simulink model "fm_demod_fixed"  (R2021b)
settings: Solver=FixedStepDiscrete  StartTime=0  StopTime=30  FixedStep=4e-06  RelTol=1e-3
libraries: dspmlti4 x1
settings Model: FPTRunName=FloatingPoint_Baseline  Creator=caccolillo  LastModifiedBy=caccolillo
settings DataIOCC: ReturnWorkspaceOutputs=off
settings DebuggingCC: SingleTaskRateTransMsg=error
settings HardwareCC: ProdBitPerPointer=32  ProdBitPerSizeT=32  ProdBitPerPtrDiffT=32  ProdLargestAtomicFloat=None  ProdIntDivRoundTo=Undefined  ProdEndianess=Unspecified  ProdWordSize=32  ProdHWDeviceType=ASIC/FPGA->ASIC/FPGA  TargetBitPerLong=64  TargetBitPerPointer=64  TargetBitPerSizeT=64  TargetBitPerPtrDiffT=64  TargetLongLongMode=on  TargetIntDivRoundTo=Zero  TargetEndianess=LittleEndian  TargetWordSize=64  TargetHWDeviceType=Custom Processor->MATLAB Host Computer  ProdEqTarget=off

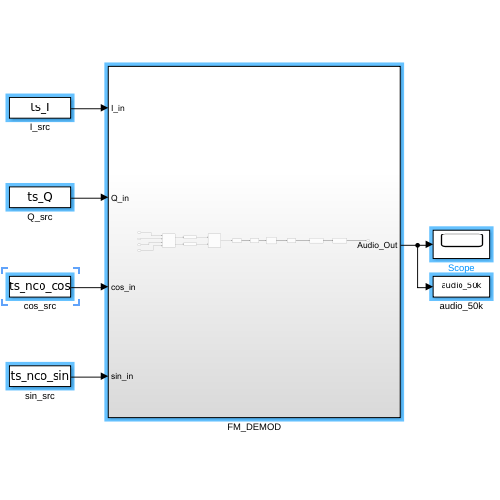
[thumbnail: Simulink's stored preview of the top-level diagram]
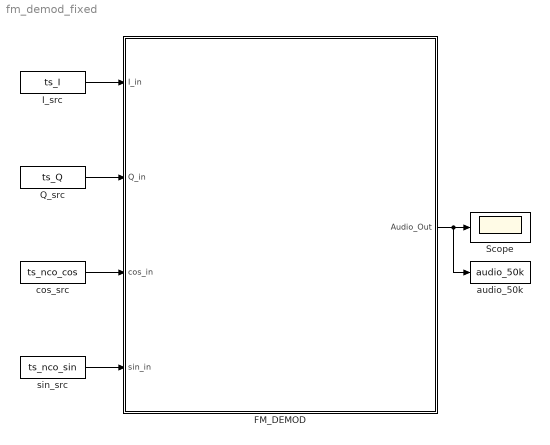
== system fm_demod_fixed ==
  FM_DEMOD : Subsystem
  I_src : FromWorkspace  VariableName=ts_I  OutDataTypeStr=fixdt(1,16,15)  SampleTime=4e-06  Interpolate=off  OutputAfterFinalValue=Holding final value
  Q_src : FromWorkspace  VariableName=ts_Q  OutDataTypeStr=fixdt(1,16,15)  SampleTime=4e-06  Interpolate=off  OutputAfterFinalValue=Holding final value
  Scope : Scope
  audio_50k : ToWorkspace  VariableName=audio_50k  SampleTime=2e-05
  cos_src : FromWorkspace  VariableName=ts_nco_cos  OutDataTypeStr=fixdt(1,16,15)  SampleTime=4e-06  Interpolate=off  OutputAfterFinalValue=Holding final value
  sin_src : FromWorkspace  VariableName=ts_nco_sin  OutDataTypeStr=fixdt(1,16,15)  SampleTime=4e-06  Interpolate=off  OutputAfterFinalValue=Holding final value
  wires:
  FM_DEMOD/1(Audio_Out) -> audio_50k/1, Scope/1
  I_src/1 -> FM_DEMOD/1(I_in)
  Q_src/1 -> FM_DEMOD/2(Q_in)
  sin_src/1 -> FM_DEMOD/4(sin_in)
  cos_src/1 -> FM_DEMOD/3(cos_in)

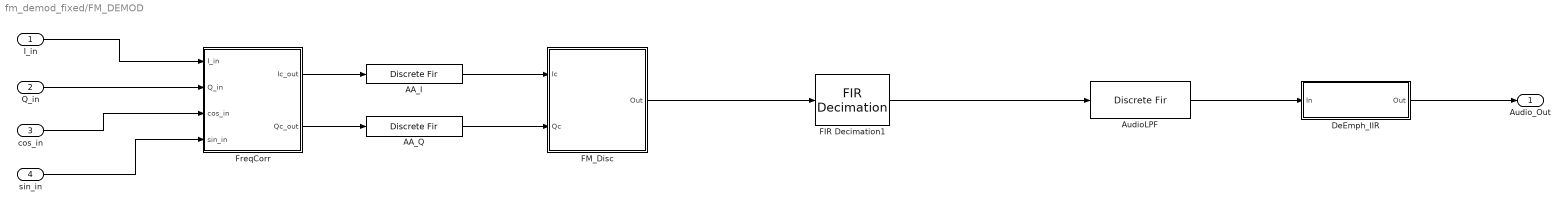
== system fm_demod_fixed/FM_DEMOD ==
  I_in : Inport
  Q_in : Inport  Port=2
  cos_in : Inport  Port=3
  sin_in : Inport  Port=4
  AA_I : DiscreteFir  Coefficients=[-6.83735984948204e-06 1.75449332456455e-05 -2.57498904954935e-05 2.22172761459078e-05 -2.99370071174519e-19 -3.92649348170435e-05 8.15857314818403e-05 -0.000102971543129532 7.91656098368774e-05 -3.24330107466436e-18 -0.000118229493833425 0.000230339323629204 -0.000275024861244747 0.000201424428805084 -1.97573802370049e-18 -0.000277296850682596 0.000521831881485624 -0.000603748721149827 0.000429629869716551 -3.69375267985403e-18 -0.00056213481227273 0.00103420375089876 -0.00117166952626484 0.000817594936231136 -6.1350079045508e-18 -0.00103254111923509 0.00186942750628691 -0.0020862979168 0.00143542734292027 -9.30071338109499e-18 -0.00176688426495698 0.00316197088837946 -0.00349061204586083 0.00237738739067954 -1.30795303176458e-17 -0.00287369810390145 0.00510160254853362 -0.00559079244160399 0.0037827464698203 -1.724148644289e-17 -0.00452266933996601 0.00799466321850092 -0.00873128617137548 0.0058928045310547 -2.14546833372083e-17 -0.00703185352755392 0.0124399916379781 -0.0136155611823128 0.00922338626974311 -2.53243457513243e-17 -0.0111510442447546 0.0199262698383597 -0.0220945427009549 0.0152176990921621 -2.84485240246462e-17 -0.0192996698147462 0.0356852825814448 -0.0413494048380904 0.0301723992042311 -3.04804610369061e-17 -0.0460953947614038 0.100083939525413 -0.150813546567284 0.186927410503456 0.800001561488201 0.186927410503456 -0.150813546567284 0.100083939525413 -0.0460953947614038 -3.04804610369061e-17 0.0301723992042311 -0.0413494048380904 0.0356852825814448 -0.0192996698147462 -2.84485240246462e-17 0.0152176990921621 -0.0220945427009549 0.0199262698383597 -0.0111510442447546 -2.53243457513243e-17 0.00922338626974311 -0.0136155611823128 0.0124399916379781 -0.00703185352755392 -2.14546833372083e-17 0.0058928045310547 -0.00873128617137548 0.00799466321850092 -0.00452266933996601 -1.724148644289e-17 0.0037827464698203 -0.00559079244160399 0.00510160254853362 -0.00287369810390145 -1.30795303176458e-17 0.00237738739067954 -0.00349061204586083 0.00316197088837946 -0.00176688426495698 -9.30071338109499e-18 0.00143542734292027 -0.0020862979168 0.00186942750628691 -0.00103254111923509 -6.1350079045508e-18 0.000817594936231136 -0.00117166952626484 0.00103420375089876 -0.00056213481227273 -3.69375267985403e-18 0.000429629869716551 -0.000603748721149827 0.000521831881485624 -0.000277296850682596 -1.97573802370049e-18 0.000201424428805084 -0.000275024861244747 0.000230339323629204 -0.000118229493833425 -3.24330107466436e-18 7.91656098368774e-05 -0.000102971543129532 8.15857314818403e-05 -3.92649348170435e-05 -2.99370071174519e-19 2.22172761459078e-05 -2.57498904954935e-05 1.75449332456455e-05 -6.83735984948204e-06]  SampleTime=4e-06  CoefDataTypeStr=fixdt(1,32,30)  OutDataTypeStr=fixdt(1,18,17)  SaturateOnIntegerOverflow=on
  AA_Q : DiscreteFir  Coefficients=[-6.83735984948204e-06 1.75449332456455e-05 -2.57498904954935e-05 2.22172761459078e-05 -2.99370071174519e-19 -3.92649348170435e-05 8.15857314818403e-05 -0.000102971543129532 7.91656098368774e-05 -3.24330107466436e-18 -0.000118229493833425 0.000230339323629204 -0.000275024861244747 0.000201424428805084 -1.97573802370049e-18 -0.000277296850682596 0.000521831881485624 -0.000603748721149827 0.000429629869716551 -3.69375267985403e-18 -0.00056213481227273 0.00103420375089876 -0.00117166952626484 0.000817594936231136 -6.1350079045508e-18 -0.00103254111923509 0.00186942750628691 -0.0020862979168 0.00143542734292027 -9.30071338109499e-18 -0.00176688426495698 0.00316197088837946 -0.00349061204586083 0.00237738739067954 -1.30795303176458e-17 -0.00287369810390145 0.00510160254853362 -0.00559079244160399 0.0037827464698203 -1.724148644289e-17 -0.00452266933996601 0.00799466321850092 -0.00873128617137548 0.0058928045310547 -2.14546833372083e-17 -0.00703185352755392 0.0124399916379781 -0.0136155611823128 0.00922338626974311 -2.53243457513243e-17 -0.0111510442447546 0.0199262698383597 -0.0220945427009549 0.0152176990921621 -2.84485240246462e-17 -0.0192996698147462 0.0356852825814448 -0.0413494048380904 0.0301723992042311 -3.04804610369061e-17 -0.0460953947614038 0.100083939525413 -0.150813546567284 0.186927410503456 0.800001561488201 0.186927410503456 -0.150813546567284 0.100083939525413 -0.0460953947614038 -3.04804610369061e-17 0.0301723992042311 -0.0413494048380904 0.0356852825814448 -0.0192996698147462 -2.84485240246462e-17 0.0152176990921621 -0.0220945427009549 0.0199262698383597 -0.0111510442447546 -2.53243457513243e-17 0.00922338626974311 -0.0136155611823128 0.0124399916379781 -0.00703185352755392 -2.14546833372083e-17 0.0058928045310547 -0.00873128617137548 0.00799466321850092 -0.00452266933996601 -1.724148644289e-17 0.0037827464698203 -0.00559079244160399 0.00510160254853362 -0.00287369810390145 -1.30795303176458e-17 0.00237738739067954 -0.00349061204586083 0.00316197088837946 -0.00176688426495698 -9.30071338109499e-18 0.00143542734292027 -0.0020862979168 0.00186942750628691 -0.00103254111923509 -6.1350079045508e-18 0.000817594936231136 -0.00117166952626484 0.00103420375089876 -0.00056213481227273 -3.69375267985403e-18 0.000429629869716551 -0.000603748721149827 0.000521831881485624 -0.000277296850682596 -1.97573802370049e-18 0.000201424428805084 -0.000275024861244747 0.000230339323629204 -0.000118229493833425 -3.24330107466436e-18 7.91656098368774e-05 -0.000102971543129532 8.15857314818403e-05 -3.92649348170435e-05 -2.99370071174519e-19 2.22172761459078e-05 -2.57498904954935e-05 1.75449332456455e-05 -6.83735984948204e-06]  SampleTime=4e-06  CoefDataTypeStr=fixdt(1,32,30)  OutDataTypeStr=fixdt(1,18,17)  SaturateOnIntegerOverflow=on
  AudioLPF : DiscreteFir  Coefficients=[1.10630118570443e-05 -1.08432976692692e-05 -1.59142086028176e-05 3.59480844718192e-05 -2.24526157623805e-19 -6.3531604158573e-05 5.04224416038869e-05 6.36395179157821e-05 -0.000128091851178763 8.0856679998092e-20 0.000191298150298555 -0.000142356645994619 -0.000169973655366647 0.00032590954596866 -4.34759523472029e-18 -0.000448672940221937 0.000322507834315517 0.000373134910757946 -0.0006951514104051 5.74683897466055e-18 0.000909547578353881 -0.000639169095981201 -0.00072412708930962 0.00132288817217507 -4.60122732508374e-18 -0.00167067624001808 0.00115536255612823 0.00128939500777255 -0.00232255579115897 -2.66068793726318e-18 0.00285886102290262 -0.00195419333229843 -0.00215730347509865 0.00384666968989025 -9.80958675736531e-18 -0.00464971230078449 0.00315294417194669 0.00345527827337028 -0.00612057431070915 3.79397487923056e-17 0.00731778722123629 -0.00494094288248589 -0.00539619807418157 0.00953469874826618 -1.60909124744493e-17 -0.0113777072824711 0.00768828985811575 0.00841482727616552 -0.0149236597035326 1.89931412434575e-17 0.0180426564366787 -0.0123150354732263 -0.0136550934687819 0.0246226012963577 -2.13362603825508e-17 -0.0312273276085871 0.0220545804321383 0.025555178741863 -0.0488196639492607 2.28602036682186e-17 0.0745834518040139 -0.0618548918364519 -0.0932073183232599 0.302453023437542 0.599997441258177 0.302453023437542 -0.0932073183232599 -0.0618548918364519 0.0745834518040139 2.28602036682186e-17 -0.0488196639492607 0.025555178741863 0.0220545804321383 -0.0312273276085871 -2.13362603825508e-17 0.0246226012963577 -0.0136550934687819 -0.0123150354732263 0.0180426564366787 1.89931412434575e-17 -0.0149236597035326 0.00841482727616552 0.00768828985811575 -0.0113777072824711 -1.60909124744493e-17 0.00953469874826618 -0.00539619807418157 -0.00494094288248589 0.00731778722123629 3.79397487923056e-17 -0.00612057431070915 0.00345527827337028 0.00315294417194669 -0.00464971230078449 -9.80958675736531e-18 0.00384666968989025 -0.00215730347509865 -0.00195419333229843 0.00285886102290262 -2.66068793726318e-18 -0.00232255579115897 0.00128939500777255 0.00115536255612823 -0.00167067624001808 -4.60122732508374e-18 0.00132288817217507 -0.00072412708930962 -0.000639169095981201 0.000909547578353881 5.74683897466055e-18 -0.0006951514104051 0.000373134910757946 0.000322507834315517 -0.000448672940221937 -4.34759523472029e-18 0.00032590954596866 -0.000169973655366647 -0.000142356645994619 0.000191298150298555 8.0856679998092e-20 -0.000128091851178763 6.36395179157821e-05 5.04224416038869e-05 -6.3531604158573e-05 -2.24526157623805e-19 3.59480844718192e-05 -1.59142086028176e-05 -1.08432976692692e-05 1.10630118570443e-05]  SampleTime=2e-05  CoefDataTypeStr=fixdt(1,32,14)  AccumDataTypeStr=fixdt(1,40,14)  OutDataTypeStr=fixdt(1,32,14)  SaturateOnIntegerOverflow=on
  DeEmph_IIR : Subsystem
  FIR Decimation1 : dspmlti4/FIR Decimation  FilterSource=Dialog parameters  h=fir1(40, 1/5)  D=5  filtStruct=Direct form transposed  FilterObject=FDECIM  framing=Enforce single-rate processing  inputOffset=0  outputBufInitCond=0  roundingMode=Floor  overflowMode=off  firstCoeffDataTypeStr=Inherit: Same word length as input  firstCoeffMin=[]  firstCoeffMax=[]  firstCoeffLastDataTypeStr=Inherit: Same word length as input  outputDataTypeStr=Inherit: Same as accumulator  outputMin=[]  outputMax=[]  outputLastDataTypeStr=Inherit: Same as accumulator
  FM_Disc : Subsystem
  FreqCorr : Subsystem
  Audio_Out : Outport
  wires:
  Q_in/1 -> FreqCorr/2(Q_in)
  FreqCorr/2(Qc_out) -> AA_Q/1
  cos_in/1 -> FreqCorr/3(cos_in)
  AA_Q/1 -> FM_Disc/2(Qc)
  sin_in/1 -> FreqCorr/4(sin_in)
  I_in/1 -> FreqCorr/1(I_in)
  FM_Disc/1(Out) -> FIR Decimation1/1
  FreqCorr/1(Ic_out) -> AA_I/1
  AA_I/1 -> FM_Disc/1(Ic)
  FIR Decimation1/1 -> AudioLPF/1
  AudioLPF/1 -> DeEmph_IIR/1(In)
  DeEmph_IIR/1(Out) -> Audio_Out/1

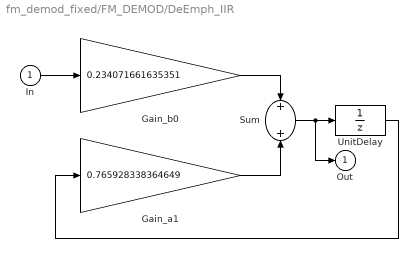
== system fm_demod_fixed/FM_DEMOD/DeEmph_IIR ==
  In : Inport
  Gain_a1 : Gain  Gain=0.765928338364649  OutDataTypeStr=fixdt(1,32,13)  SaturateOnIntegerOverflow=on  SampleTime=2e-5
  Gain_b0 : Gain  Gain=0.234071661635351  OutDataTypeStr=fixdt(1,32,13)  SaturateOnIntegerOverflow=on  SampleTime=2e-5
  Sum : Sum  OutDataTypeStr=fixdt(1,32,13)  SaturateOnIntegerOverflow=on  SampleTime=2e-5
  UnitDelay : UnitDelay  SampleTime=2e-5
  Out : Outport
  wires:
  Sum/1 -> Out/1, UnitDelay/1
  In/1 -> Gain_b0/1
  Gain_a1/1 -> Sum/2
  Gain_b0/1 -> Sum/1
  UnitDelay/1 -> Gain_a1/1

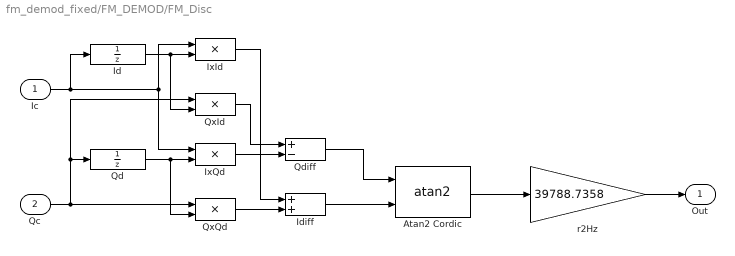
== system fm_demod_fixed/FM_DEMOD/FM_Disc ==
  Ic : Inport
  Qc : Inport  Port=2
  Atan2 Cordic : Trigonometry  Operator=atan2  ApproximationMethod=CORDIC
  Id : UnitDelay  SampleTime=4e-06  HasFrameUpgradeWarning=on
  Idiff : Sum  OutDataTypeStr=fixdt(1,18,14)  RndMeth=Round  SaturateOnIntegerOverflow=on
  IxId : Product  OutDataTypeStr=fixdt(1,18,14)  RndMeth=Round  SaturateOnIntegerOverflow=on
  IxQd : Product  OutDataTypeStr=fixdt(1,18,14)  RndMeth=Round  SaturateOnIntegerOverflow=on
  Qd : UnitDelay  SampleTime=4e-06  HasFrameUpgradeWarning=on
  Qdiff : Sum  Inputs=+-  OutDataTypeStr=fixdt(1,18,14)  RndMeth=Round  SaturateOnIntegerOverflow=on
  QxId : Product  OutDataTypeStr=fixdt(1,18,14)  RndMeth=Round  SaturateOnIntegerOverflow=on
  QxQd : Product  OutDataTypeStr=fixdt(1,18,14)  RndMeth=Round  SaturateOnIntegerOverflow=on
  r2Hz : Gain  Gain=39788.7358  OutDataTypeStr=fixdt(1,32,14)  RndMeth=Round  SaturateOnIntegerOverflow=on
  Out : Outport
  wires:
  Ic/1 -> IxQd/1, IxId/1, Id/1
  Qc/1 -> Qd/1, QxId/1, QxQd/1
  Id/1 -> QxId/2, IxId/2
  QxId/1 -> Qdiff/1
  Qd/1 -> IxQd/2, QxQd/2
  Atan2 Cordic/1 -> r2Hz/1
  r2Hz/1 -> Out/1
  Idiff/1 -> Atan2 Cordic/2
  Qdiff/1 -> Atan2 Cordic/1
  IxQd/1 -> Qdiff/2
  QxQd/1 -> Idiff/2
  IxId/1 -> Idiff/1

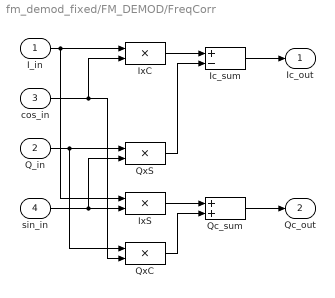
== system fm_demod_fixed/FM_DEMOD/FreqCorr ==
  I_in : Inport
  Q_in : Inport  Port=2
  cos_in : Inport  Port=3
  sin_in : Inport  Port=4
  Ic_sum : Sum  Inputs=+-  OutDataTypeStr=fixdt(1,18,17)  RndMeth=Round  SaturateOnIntegerOverflow=on
  IxC : Product  OutDataTypeStr=fixdt(1,18,17)  RndMeth=Round  SaturateOnIntegerOverflow=on
  IxS : Product  OutDataTypeStr=fixdt(1,18,17)  RndMeth=Round  SaturateOnIntegerOverflow=on
  Qc_sum : Sum  OutDataTypeStr=fixdt(1,18,17)  RndMeth=Round  SaturateOnIntegerOverflow=on
  QxC : Product  OutDataTypeStr=fixdt(1,18,17)  RndMeth=Round  SaturateOnIntegerOverflow=on
  QxS : Product  OutDataTypeStr=fixdt(1,18,17)  RndMeth=Round  SaturateOnIntegerOverflow=on
  Ic_out : Outport
  Qc_out : Outport  Port=2
  wires:
  I_in/1 -> IxC/1, IxS/1
  cos_in/1 -> IxC/2, QxC/2
  Q_in/1 -> QxS/1, QxC/1
  sin_in/1 -> QxS/2, IxS/2
  Ic_sum/1 -> Ic_out/1
  Qc_sum/1 -> Qc_out/1
  IxS/1 -> Qc_sum/1
  QxC/1 -> Qc_sum/2
  QxS/1 -> Ic_sum/2
  IxC/1 -> Ic_sum/1
